simulink model "single_phase_to_3phase"  (R2025a)
settings: Solver=ode23tb  StartTime=0.0  StopTime=10.0  RelTol=1e-3  EnableMultiTasking=on
undefined symbols (not defined in the file): DiscIntNeverNeededParam, LowerLimit, UpperLimit, Vsrc_amp
libraries: powerlib_extras x8, spsVoltageMeasurementLib x7, spsGroundLib x5, spsSeriesRLCBranchLib x4, spsThreePhaseSeriesRLCBranchLib x2, spsUniversalBridgeLib x2, spsACVoltageSourceLib x1, simulink x1, spsThreePhaseSeriesRLCLoadLib x1, spsThreePhaseVIMeasurementLib x1, spspowerguiLib x1
settings Model: Creator=DELL  LastModifiedBy=SimuVerity Contributors
settings SolverCC: ZeroCrossAlgorithm=Non-adaptive  AlgebraicLoopSolver=TrustRegion
settings DataIOCC: LimitDataPoints=on  SaveFormat=Array  SignalLoggingSaveFormat=ModelDataLogs  ReturnWorkspaceOutputs=off
settings OptimizationCC: ExpressionDepthLimit=2147483647.0  InitFltsAndDblsToZero=on  LifeSpan=inf
settings DebuggingCC: UnderspecifiedInitializationDetection=Classic  MergeDetectMultiDrivingBlocksExec=none  SolverPrmCheckMsg=warning  FcnCallInpInsideContextMsg=warning  UnconnectedInputMsg=warning  UnconnectedOutputMsg=warning  UnconnectedLineMsg=warning  StateNameClashWarn=warning  SFUnexpectedBacktrackingDiag=warning  SFNoUnconditionalDefaultTransitionDiag=warning  SFExecutionAtInitializationDiag=none  ArithmeticOperatorsInVariantConditions=warning
settings HardwareCC: ProdBitPerPointer=32.0  ProdBitPerSizeT=32.0  ProdBitPerPtrDiffT=32.0  ProdLargestAtomicFloat=None  ProdIntDivRoundTo=Undefined  ProdEndianess=Unspecified  ProdWordSize=32.0  ProdHWDeviceType=32-bit Generic
settings ModelReferenceCC: PropagateSignalLabelsOutOfModel=off
settings RTWCC: GPUComputeCapability=3.5
settings CodeAppCC: StateflowObjectComments=on
settings GRTTargetCC: TargetLangStandard=C89/C90 (ANSI)  CombineOutputUpdateFcns=off  GRTInterface=on
settings ConfigComp: CovMetricSettings=dw  CovSaveCumulativeToWorkspaceVar=on  CovSaveSingleToWorkspaceVar=on

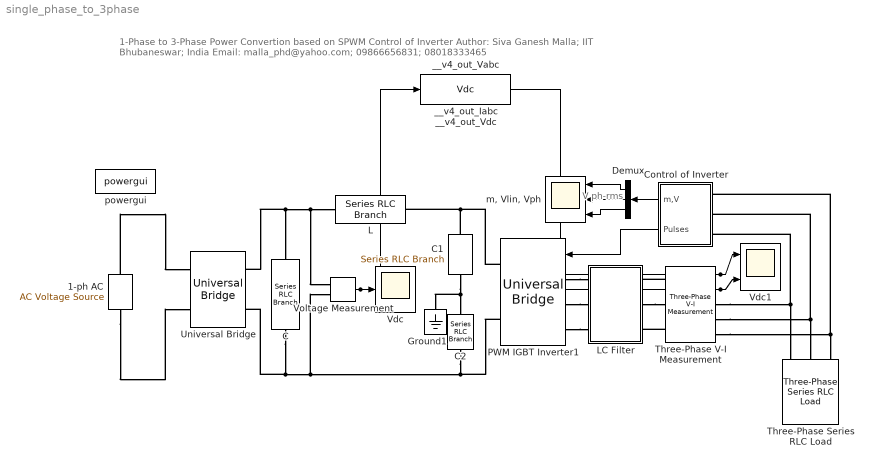
== system single_phase_to_3phase ==
  note: V ph-rms
  note: 1-Phase to 3-Phase Power Convertion based on SPWM Control of Inverter
      | Author: Siva Ganesh Malla; IIT Bhubaneswar; India
      | Email: malla_phd@yahoo.com; 09866656831; 08018333465
  1-ph AC : spsACVoltageSourceLib/AC Voltage Source  Amplitude=Vsrc_amp  Phase=0  Frequency=50  SampleTime=0.00001  Measurements=None  BusType=swing  Pref=10e3  Qref=0  Qmin=-inf  Qmax=+inf
  C : spsSeriesRLCBranchLib/Series RLC Branch  LConnTagsString=__new0  RConnTagsString=__new0  BranchType=C  Resistance=1  Inductance=1e-3  SetiL0=off  InitialCurrent=0  Capacitance=10e-6  Setx0=off  InitialVoltage=0  Measurements=None
  C1 : spsSeriesRLCBranchLib/Series RLC Branch  LConnTagsString=__new0  RConnTagsString=__new0  BranchType=C  Resistance=1  Inductance=1e-3  SetiL0=off  InitialCurrent=0  Capacitance=2300e-6  Setx0=off  InitialVoltage=0  Measurements=None
  C2 : spsSeriesRLCBranchLib/Series RLC Branch  LConnTagsString=__new0  RConnTagsString=__new0  BranchType=C  Resistance=1  Inductance=1e-3  SetiL0=off  InitialCurrent=0  Capacitance=2300e-6  Setx0=off  InitialVoltage=0  Measurements=None
  Control of Inverter : Subsystem
  Demux : Demux  Outputs=3
  Ground1 : spsGroundLib/Ground  LConnTagsString=a
  L : spsSeriesRLCBranchLib/Series RLC Branch  LConnTagsString=__new0  RConnTagsString=__new0  BranchType=L  Resistance=1  Inductance=0.1e-3  SetiL0=off  InitialCurrent=0  Capacitance=1e-6  Setx0=off  InitialVoltage=0  Measurements=None
  LC Filter : Subsystem
  PWM IGBT Inverter1 : spsUniversalBridgeLib/Universal Bridge  Arms=3  SnubberResistance=5000  SnubberCapacitance=inf  Device=GTO / Diodes  Ron=1e-3  Lon=0  ForwardVoltages="[  0.0  0.0  ]"  ForwardVoltage=.8  GTOparameters=[ 1e-6 ,1e-6 ]  IGBTparameters=[ 1e-6 , 2e-6 ]  Measurements=Device currents  Measurements_2=None  converterType=Rectifier
      settings: AttributesFormatString=\n
  Three-Phase Series RLC Load : spsThreePhaseSeriesRLCLoadLib/Three-Phase Series RLC Load  LConnTagsString=A|B|C  Configuration=Y (grounded)  NominalVoltage=400  Vabc=[1e3 1e3 1e3]  Vabcp=[1e3 1e3 1e3]  NominalFrequency=50  UnbalancedPower=off  ActivePower=P_load  InductivePower=0  CapacitivePower=0  Pabc=[10e3 9e3 11e3]  QLabc=[100 90 110]  QCabc=[100 90 110]  Pabcp=[10e3 9e3 11e3]  QLabcp=[100 90 110]  QCabcp=[100 90 110]  Measurements=None  LoadType=constant Z
  Three-Phase V-I Measurement : spsThreePhaseVIMeasurementLib/Three-Phase V-I Measurement  VoltageMeasurement=phase-to-ground  SetLabelV=off  LabelV=Vabc  Vpu=off  VpuLL=off  CurrentMeasurement=yes  SetLabelI=off  LabelI=Iabc  Ipu=off  Pbase=100e6  Vbase=500e3  OutputType=Complex  PhasorSimulation=off  PSBequivalent=0
  Universal Bridge : spsUniversalBridgeLib/Universal Bridge  Arms=2  SnubberResistance=1e5  SnubberCapacitance=inf  Device=Diodes  Ron=1e-3  Lon=0  ForwardVoltages="[  0  0  ]"  ForwardVoltage=0  GTOparameters=[ 10e-6 , 20e-6 ]  IGBTparameters=[ 1e-6 , 2e-6 ]  Measurements=None  Measurements_2=None  converterType=Rectifier
  Vdc : Scope
      settings: SampleTime=100e-6  TimeSpan=1  ActiveDisplayYMinimum=475  ActiveDisplayYMaximum=675  DataLoggingVariableName=Ia_1
  Vdc1 : Scope  NumInputPorts=2
      settings: SampleTime=100e-6  TimeSpan=1  ActiveDisplayYMinimum=-350  ActiveDisplayYMaximum=350  DataLoggingVariableName=Ia_2
  Voltage Measurement : spsVoltageMeasurementLib/Voltage Measurement  PhasorSimulation=off  OutputType=Complex  PSBequivalent=0
  __v4_out_Iabc : ToWorkspace  VariableName=Iabc  SaveFormat=Timeseries  SampleTime=-1
  __v4_out_Vabc : ToWorkspace  VariableName=Vabc  SaveFormat=Timeseries  SampleTime=-1
  __v4_out_Vdc : ToWorkspace  VariableName=Vdc  SaveFormat=Timeseries  SampleTime=-1
  "m, Vlin, Vph" : Scope  NumInputPorts=3
      settings: SampleTime=100e-6  TimeSpan=1  ActiveDisplayYMinimum=0.93  ActiveDisplayYMaximum=0.995  DataLoggingVariableName=Ia_
  powergui : spspowerguiLib/powergui  SimulationMode=Discrete  SampleTime=50e-6  frequency=60  Iterations=50  frequencyindice=0  Pbase=100e6  ErrMax=1e-4  UnitsV=kV  UnitsW=MW  buscounter=0  FunctionMessages=off  echomessages=off  EnableUseOfTLC=off  CurrentSourceSwitches=off  DisableSnubberDevices=off  DisableRonSwitches=off  DisableVfSwitches=off  DisplayEquations=off  AutomaticDiscreteSolvers=off  SolverType=Tustin/Backward Euler (TBE)  Interpol=off  ExternalGateDelay=off  methode=off  Ts=0  x0status=blocks  SPID=off  SwTol=0  HookPort=off  NonlinearTolerance=1e-4  nMaxIteration=100  ContinueOnMaxIteration=off  RestoreLinks=warning  ResistiveCurrentMeasurement=off  Frange=[0:2:500]  Ylog=off  Xlog=on  ShowGrid=off  save=off  variable=ZData  structure=0  ZoomFFT=on  StartTime=0.0  cycles=1  DisplayStyle=1  fundamental=60  FreqAxis=off  MaxFrequency=1000  frequencyindicesteady=1  RmsSteady=1  display=off
  wires:
  Control of Inverter/2(Pulses) -> PWM IGBT Inverter1/1
  Control of Inverter/1(m,V) -> Demux/1
  Demux/1 -> "m, Vlin, Vph"/1
  Demux/2 -> "m, Vlin, Vph"/2
  Demux/3 -> "m, Vlin, Vph"/3
  Voltage Measurement/1 -> Vdc/1, __v4_out_Vdc/1
  Three-Phase V-I Measurement/1 -> Vdc1/1, __v4_out_Vabc/1
  Three-Phase V-I Measurement/2 -> Vdc1/2, __v4_out_Iabc/1
  connections:
  1-ph AC/RConn1 -- Universal Bridge/LConn1
  1-ph AC/LConn1 -- Universal Bridge/LConn2
  Universal Bridge/RConn1 -- C/LConn1 -- L/LConn1 -- Voltage Measurement/LConn1
  Universal Bridge/RConn2 -- C/RConn1 -- C2/RConn1 -- PWM IGBT Inverter1/RConn2 -- Voltage Measurement/LConn2
  PWM IGBT Inverter1/LConn1 -- LC Filter/LConn1
  PWM IGBT Inverter1/LConn2 -- LC Filter/LConn2
  PWM IGBT Inverter1/LConn3 -- LC Filter/LConn3
  Three-Phase V-I Measurement/RConn1 -- Three-Phase Series RLC Load/LConn1 -- Control of Inverter/LConn3
  Three-Phase V-I Measurement/RConn2 -- Three-Phase Series RLC Load/LConn2 -- Control of Inverter/LConn2
  Three-Phase V-I Measurement/RConn3 -- Three-Phase Series RLC Load/LConn3 -- Control of Inverter/LConn1
  Three-Phase V-I Measurement/LConn1 -- LC Filter/RConn1
  LC Filter/RConn2 -- Three-Phase V-I Measurement/LConn2
  Three-Phase V-I Measurement/LConn3 -- LC Filter/RConn3
  C1/LConn1 -- PWM IGBT Inverter1/RConn1 -- L/RConn1
  C1/RConn1 -- C2/LConn1 -- Ground1/LConn1

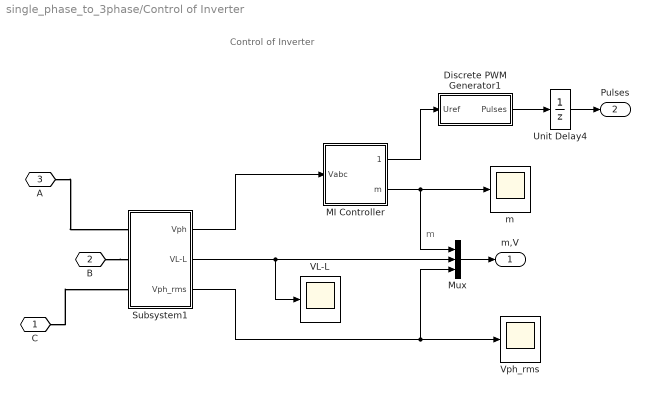
== system single_phase_to_3phase/Control of Inverter ==
  note: Control of Inverter
  note: m
  Discrete PWM Generator1 : Subsystem  AncestorBlock=|  DialogController=POWERSYS.PowerSysDialog  mask(Discrete PWM Generator){GeneratorMode=3-arm  bridge (6 pulses), Fc=4000, Ts=20e-6, Internal=off, mIndex=0.95, Freq=50, Phase=0}
      | powerlib_extras/Discrete 
      | Control Blocks/Discrete
      | PWM Generator
      mask prompts: GeneratorMode "Generator Mode"; Fc "Carrier frequency (Hz):"; Ts "Sample time:"; Internal "Internal generation of modulating signal(s)"; mIndex "Modulation index  (0<m<1) :"; Freq "Frequency of output voltage (Hz)"; Phase "Phase of output voltage (degrees)"
      mask help:
      | This discrete block generates pulses for carrier-based PWM (Pulse Width Modulation), self-commutated IGBTs,GTOs or FETs bridges.
      |
      | Depending on the number of bridge arms selected in the "Generator Mode" parameter, the block can be used either for single-phase or three-phase PWM control.
      mask init:
      | powericon('psbcallbacks',gcb,'Discrete PWM Generator');
      | if Freq==0
      |     Phase=90;
      | end
      | switch GeneratorMode
      | case 1,
      |     Internal_Phase=0;
      |    Signal_PortWidth=1;
      |    Select1_Elements=[1 2];
      |    Select1_PortWidth=2;
      |    Select3_Elements=[1 2];
      |    Select3_PortWidth=4;
      | case 2,
      |     Internal_Phase=0;
      |     Signal_PortWidth=1;
      |     Select1_Elements=[1 2];
      |     Select1_PortWidth=2;
      |     Select3_Elements=[1 2 3 4];
      |     Select3_PortWidth=4;
      | case 3,
      |     Internal_Phase=[0 -2*pi/3 2*pi/3];
      |     Signal_PortWidth=3;
      |     Select1_Elements=[1 4 2 5 3 6];
      |     Select1_PortWidth=6;
      |    Select3_Elements=[1 2 3 4 5 6];
      |    Select3_PortWidth=12;
      | case 4,
      |     Internal_Phase=[0 -2*pi/3 2*pi/3];
      |     Signal_PortWidth=3;
      |     Select1_Elements=[1 4 2 5 3 6];
      |     Select1_PortWidth=6;
      |    Select3_Elements=[1 2 3 4 5 6 7 8 9 10 11 12];
      |    Select3_PortWidth=12;
      | end
      | power_initmask();
      mask Help:
      | The output pulses are a vector (with values=0 or 1). Depending on the selected "Generator Mode", the output vector contains:
      | For a 1-arm  bridge: Two pulses. Pulse 1 is for the upper switch and pulse 2 is for the lower switch.
      | For a 2-arm  bridge: Four pulses. Pulses 1 and 3 are respectively for the upper switches of the first and second arm. Pulses 2 and 4 are for the lower switches.
      | For a 3-arm  bridge: Six pulses. Pulses 1,3 and 5 are respectively for the upper switches of the first,second and third arm. Pulses 2,4 and 6 are for the lower switches.
      | For double 3-arm bridges: Twelve pulses.The first six pulses (pulses 1 to 6) must be sent to the first 3-arm bridge and the last six (pulses 7 to 12) to the second 3-arm bridge.
      | 
      | By selecting "Internal generation" you can can control the modulation index m, frequency and phase of the output voltage  from the internal parameters (m, Freq and Phase). Otherwise, external signals are used for pulse generation. The width of the input vector must be 1 for single phase bridges ( 1-arm or 2-arm)  and 3 for 3-phase bridges  (single or double bridge).
      mask TypeOptions GeneratorMode: 1-arm  bridge (2 pulses) | 2-arm  bridge (4 pulses) | 3-arm  bridge (6 pulses) | Double 3-arm  bridges (12 pulses)
      mask Callback Internal: powericon('psbcallbacks',gcb,'Discrete PWM Generator',[]);
  MI Controller : Subsystem
  Mux : Mux  Inputs=3
  Subsystem1 : Subsystem
  Unit Delay4 : UnitDelay  SampleTime=20e-6
  VL-L : Scope
      settings: SampleTime=100e-6  TimeSpan=0.4  ActiveDisplayYMinimum=-700  ActiveDisplayYMaximum=700  DataLoggingVariableName=Vabc_line
  Vph_rms : Scope
      settings: SampleTime=100e-6  TimeSpan=0.4  ActiveDisplayYMinimum=29.5  ActiveDisplayYMaximum=33.75  DataLoggingVariableName=Vabc_rms
  m : Scope
      settings: SampleTime=100e-6  TimeSpan=0.04  ActiveDisplayYMinimum=0.7  ActiveDisplayYMaximum=1.5  DataLoggingVariableName=modulation_index
  C : PMIOPort  Side=Left
  B : PMIOPort  Port=2  Side=Left
  A : PMIOPort  Port=3  Side=Left
  m,V : Outport
  Pulses : Outport  Port=2
  wires:
  Mux/1 -> m,V/1
  MI Controller/2(m) -> m/1, Mux/1
  Unit Delay4/1 -> Pulses/1
  Discrete PWM Generator1/1(Pulses) -> Unit Delay4/1
  MI Controller/1(Vabc_inv) -> Discrete PWM Generator1/1(Uref)
  Subsystem1/1(Vph) -> MI Controller/1(Vabc)
  Subsystem1/2(VL-L) -> VL-L/1, Mux/2
  Subsystem1/3(Vph_rms) -> Vph_rms/1, Mux/3
  connections:
  A/RConn1 -- Subsystem1/LConn1
  B/RConn1 -- Subsystem1/LConn2
  C/RConn1 -- Subsystem1/LConn3

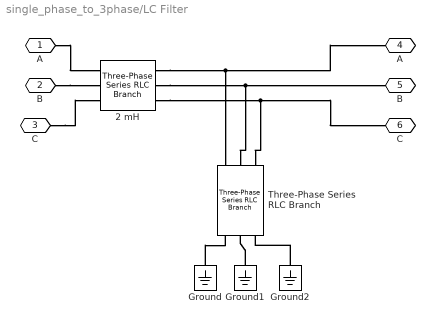
== system single_phase_to_3phase/LC Filter ==
  "2 mH " : spsThreePhaseSeriesRLCBranchLib/Three-Phase Series RLC Branch  LConnTagsString=A|B|C  RConnTagsString=A|B|C  BranchType=L  Resistance=1.0  Inductance=36e-3  Capacitance=1.0  Measurements=None
  Ground : spsGroundLib/Ground  LConnTagsString=a
  Ground1 : spsGroundLib/Ground  LConnTagsString=a
  Ground2 : spsGroundLib/Ground  LConnTagsString=a
  Three-Phase Series RLC Branch : spsThreePhaseSeriesRLCBranchLib/Three-Phase Series RLC Branch  LConnTagsString=A|B|C  RConnTagsString=A|B|C  BranchType=C  Resistance=.1  Inductance=1e-3  Capacitance=6.85e-7  Measurements=None
  A : PMIOPort  Side=Left
  B : PMIOPort  Port=2  Side=Left
  C : PMIOPort  Port=3  Side=Left
  "A " : PMIOPort  Port=4  Side=Right
  "B " : PMIOPort  Port=5  Side=Right
  "C " : PMIOPort  Port=6  Side=Right
  connections:
  B/RConn1 -- "2 mH "/LConn2
  A/RConn1 -- "2 mH "/LConn1
  C/RConn1 -- "2 mH "/LConn3
  "2 mH "/RConn1 -- "A "/RConn1 -- Three-Phase Series RLC Branch/LConn1
  "2 mH "/RConn2 -- "B "/RConn1 -- Three-Phase Series RLC Branch/LConn2
  "2 mH "/RConn3 -- "C "/RConn1 -- Three-Phase Series RLC Branch/LConn3
  Ground/LConn1 -- Three-Phase Series RLC Branch/RConn1
  Ground1/LConn1 -- Three-Phase Series RLC Branch/RConn2
  Ground2/LConn1 -- Three-Phase Series RLC Branch/RConn3

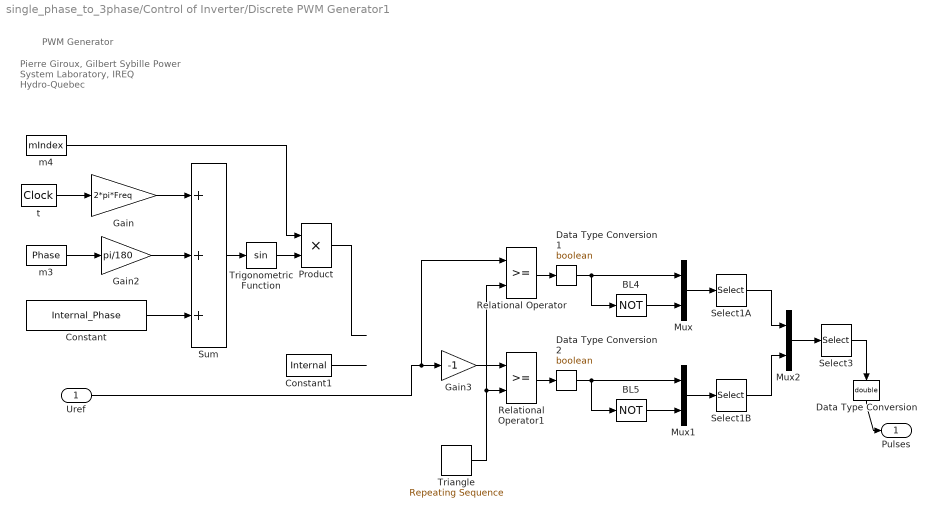
== system single_phase_to_3phase/Control of Inverter/Discrete PWM Generator1 ==
  note: Pierre Giroux, Gilbert Sybille
      | Power System Laboratory, IREQ
      | Hydro-Quebec
  note: PWM Generator
  Uref : Inport
  BL4 : Logic  Operator=NOT  Inputs=1
  BL5 : Logic  Operator=NOT  Inputs=1
  Constant : Constant  Value=Internal_Phase
  Constant1 : Constant  Value=Internal
  Data Type Conversion : DataTypeConversion  OutDataTypeStr=double
  Data Type Conversion1 : DataTypeConversion  OutDataTypeStr=boolean
  Data Type Conversion2 : DataTypeConversion  OutDataTypeStr=boolean
  Gain : Gain  Gain=2*pi*Freq  SaturateOnIntegerOverflow=on  OutDataTypeStr=Inherit: Same as input  ParamDataTypeStr=Inherit: Same as input
  Gain2 : Gain  Gain=pi/180  SaturateOnIntegerOverflow=on  OutDataTypeStr=Inherit: Same as input  ParamDataTypeStr=Inherit: Same as input
  Gain3 : Gain  Gain=-1  SaturateOnIntegerOverflow=on  OutDataTypeStr=Inherit: Same as input  ParamDataTypeStr=Inherit: Same as input
  Mux : Mux  Inputs=2
  Mux1 : Mux  Inputs=2
  Mux2 : Mux  Inputs=2
  Product : Product  InputSameDT=on  SaturateOnIntegerOverflow=on  OutDataTypeStr=Inherit: Same as first input
  Relational Operator : RelationalOperator
  Relational Operator1 : RelationalOperator
  Select1A : Selector  InputPortWidth=Select1_PortWidth  IndexOptions=Index vector (dialog)  Indices=Select1_Elements  OutputSizes=1
  Select1B : Selector  InputPortWidth=Select1_PortWidth  IndexOptions=Index vector (dialog)  Indices=Select1_Elements  OutputSizes=1
  Select3 : Selector  InputPortWidth=Select3_PortWidth  IndexOptions=Index vector (dialog)  Indices=Select3_Elements  OutputSizes=1
  Sum : Sum  Inputs=+++  InputSameDT=on  SaturateOnIntegerOverflow=on  OutDataTypeStr=Inherit: Same as first input
  Triangle : simulink/Sources/Repeating Sequence  rep_seq_t=[0 1/Fc/4 3/Fc/4 1/Fc]  rep_seq_y=[0 -1 1 0]
  Trigonometric Function : Trigonometry
  m3 : Constant  Value=Phase
  m4 : Constant  Value=mIndex
  t : DigitalClock  SampleTime=Ts
  Pulses : Outport
  wires:
  Mux2/1 -> Select3/1
  Select1B/1 -> Mux2/2
  Select1A/1 -> Mux2/1
  Mux1/1 -> Select1B/1
  Mux/1 -> Select1A/1
  BL5/1 -> Mux1/2
  BL4/1 -> Mux/2
  Gain3/1 -> Relational Operator1/1
  Triangle/1 -> Relational Operator1/2, Relational Operator/2
  Product/1 -> ?
  Constant1/1 -> ?
  Uref/1 -> Relational Operator/1, Gain3/1
  Trigonometric Function/1 -> Product/2
  Sum/1 -> Trigonometric Function/1
  m4/1 -> Product/1
  Constant/1 -> Sum/3
  m3/1 -> Gain2/1
  Gain2/1 -> Sum/2
  Gain/1 -> Sum/1
  t/1 -> Gain/1
  Select3/1 -> Data Type Conversion/1
  Data Type Conversion/1 -> Pulses/1
  Relational Operator/1 -> Data Type Conversion1/1
  Data Type Conversion1/1 -> BL4/1, Mux/1
  Relational Operator1/1 -> Data Type Conversion2/1
  Data Type Conversion2/1 -> BL5/1, Mux1/1

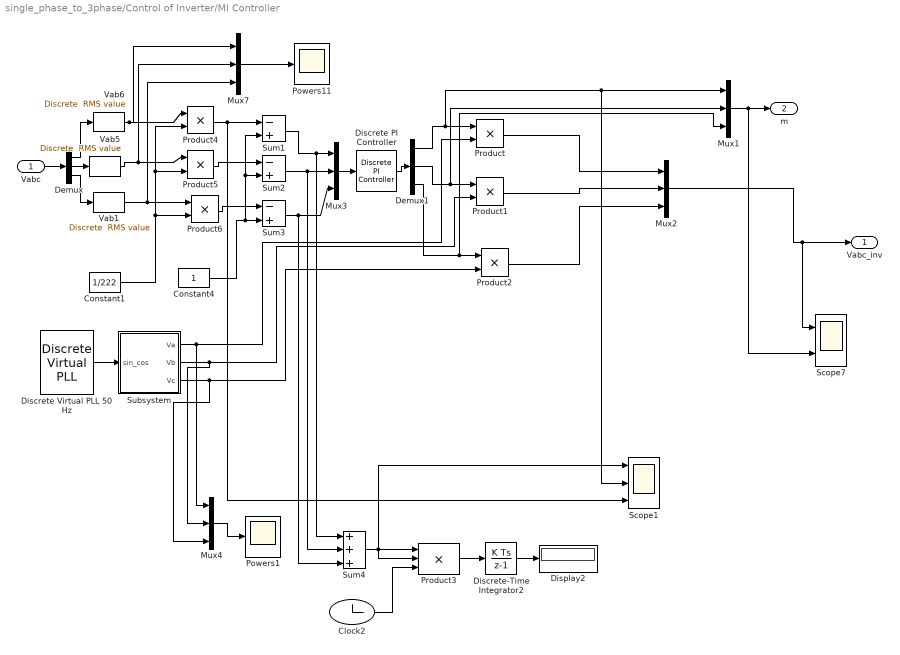
== system single_phase_to_3phase/Control of Inverter/MI Controller ==
  Vabc : Inport
  Clock2 : Clock
  Constant1 : Constant  Value=1/222
  Constant4 : Constant
  Demux : Demux  Outputs=3
  Demux1 : Demux  Outputs=3
  Discrete PI Controller : powerlib_extras/Discrete  Control Blocks/Discrete PI Controller  Kp=1.6  Ki=36  Par_Limits=[1.2 -1]  Init=0  Ts=20e-6
  Discrete Virtual PLL 50 Hz : powerlib_extras/Discrete  Control Blocks/Discrete Virtual PLL  Freq=50  Phase=0  Ts=20e-6
  Discrete-Time Integrator2 : DiscreteIntegrator  SampleTime=20e-6  UpperSaturationLimit=UpperLimit  LowerSaturationLimit=LowerLimit  ICPrevOutput=DiscIntNeverNeededParam  ICPrevScaledInput=DiscIntNeverNeededParam
  Display2 : Display
  Mux{1..4,7} (5 alike) : Mux  Inputs=3
  Powers1 : Scope
      settings: SampleTime=100e-6  ActiveDisplayYMinimum=-1  ActiveDisplayYMaximum=1  DataLoggingVariableName=ScopeData3
  Powers11 : Scope
      settings: SampleTime=100e-6  ActiveDisplayYMinimum=452  ActiveDisplayYMaximum=465  DataLoggingVariableName=ScopeData6
  Product{,1..2,4..6} (6 alike) : Product  RndMeth=Zero
  Product3 : Product  Inputs=3  InputSameDT=on  RndMeth=Zero  SaturateOnIntegerOverflow=on  OutDataTypeStr=Inherit: Same as first input
  Scope1 : Scope  NumInputPorts=3
      settings: TimeSpan=0.1  ActiveDisplayYMinimum=-0.005  ActiveDisplayYMaximum=0.0175  DataLoggingVariableName=psbbridges_str6
  Scope7 : Scope  NumInputPorts=2
      settings: TimeSpan=0.1  ActiveDisplayYMinimum=-1.1  ActiveDisplayYMaximum=1.1  DataLoggingVariableName=psbbridges_str2
  Subsystem : Subsystem
  Sum1 : Sum  Inputs=-+  InputSameDT=on  SaturateOnIntegerOverflow=on  OutDataTypeStr=Inherit: Same as first input
  Sum2 : Sum  Inputs=-+  InputSameDT=on  SaturateOnIntegerOverflow=on  OutDataTypeStr=Inherit: Same as first input
  Sum3 : Sum  Inputs=-+  InputSameDT=on  SaturateOnIntegerOverflow=on  OutDataTypeStr=Inherit: Same as first input
  Sum4 : Sum  Inputs=+++  InputSameDT=on  SaturateOnIntegerOverflow=on  OutDataTypeStr=Inherit: Same as first input
  Vab1 : powerlib_extras/Discrete Measurements/Discrete  RMS value  Freq=50  Mag_Init=0  Ts=20e-6
  Vab5 : powerlib_extras/Discrete Measurements/Discrete  RMS value  Freq=50  Mag_Init=0  Ts=20e-6
  Vab6 : powerlib_extras/Discrete Measurements/Discrete  RMS value  Freq=50  Mag_Init=0  Ts=20e-6
  Vabc_inv : Outport
  m : Outport  Port=2
  wires:
  Mux2/1 -> Vabc_inv/1, Scope7/1
  Product/1 -> Mux2/1
  Product1/1 -> Mux2/2
  Product2/1 -> Mux2/3
  Mux1/1 -> m/1, Scope7/2
  Vab5/1 -> Mux7/2, Product5/1
  Vab1/1 -> Mux7/3, Product6/1
  Constant4/1 -> Sum3/2, Sum2/2, Sum1/2
  Sum1/1 -> Mux3/1, Sum4/1
  Vabc/1 -> Demux/1
  Demux/1 -> Vab6/1
  Demux/2 -> Vab5/1
  Demux/3 -> Vab1/1
  Product3/1 -> Discrete-Time Integrator2/1
  Clock2/1 -> Product3/3
  Discrete-Time Integrator2/1 -> Display2/1
  Sum2/1 -> Mux3/2, Sum4/2
  Sum3/1 -> Mux3/3, Sum4/3
  Mux3/1 -> Discrete PI Controller/1
  Discrete PI Controller/1 -> Demux1/1
  Demux1/1 -> Product/1, Mux1/1, Scope1/2
  Demux1/2 -> Product1/1, Mux1/2
  Demux1/3 -> Product2/1, Mux1/3
  Product4/1 -> Sum1/1, Scope1/3
  Product5/1 -> Sum2/1
  Product6/1 -> Sum3/1
  Vab6/1 -> Mux7/1, Product4/1
  Mux7/1 -> Powers11/1
  Discrete Virtual PLL 50 Hz/2 -> Subsystem/1(sin_cos)
  Subsystem/1(Va) -> Product/2, Mux4/1
  Subsystem/2(Vb) -> Product1/2, Mux4/2
  Subsystem/3(Vc) -> Product2/2, Mux4/3
  Mux4/1 -> Powers1/1
  Constant1/1 -> Product6/2, Product5/2, Product4/2
  Sum4/1 -> Product3/1, Product3/2, Scope1/1

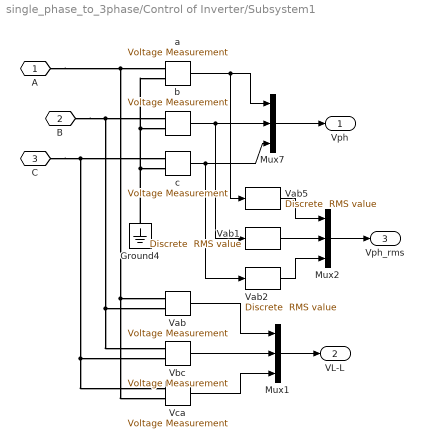
== system single_phase_to_3phase/Control of Inverter/Subsystem1 ==
  Ground4 : spsGroundLib/Ground  LConnTagsString=a
  Mux1 : Mux  Inputs=3
  Mux2 : Mux  Inputs=3
  Mux7 : Mux  Inputs=3
  Vab : spsVoltageMeasurementLib/Voltage Measurement  Tag=PoWeRsYsTeMmEaSuReMeNt  PhasorSimulation=off  OutputType=Magnitude  PSBequivalent=0
  Vab1 : powerlib_extras/Discrete Measurements/Discrete  RMS value  Freq=50  Mag_Init=0  Ts=20e-6
  Vab2 : powerlib_extras/Discrete Measurements/Discrete  RMS value  Freq=50  Mag_Init=0  Ts=20e-6
  Vab5 : powerlib_extras/Discrete Measurements/Discrete  RMS value  Freq=50  Mag_Init=0  Ts=20e-6
  Vbc : spsVoltageMeasurementLib/Voltage Measurement  Tag=PoWeRsYsTeMmEaSuReMeNt  PhasorSimulation=off  OutputType=Magnitude  PSBequivalent=0
  Vca : spsVoltageMeasurementLib/Voltage Measurement  Tag=PoWeRsYsTeMmEaSuReMeNt  PhasorSimulation=off  OutputType=Magnitude  PSBequivalent=0
  a : spsVoltageMeasurementLib/Voltage Measurement  Tag=PoWeRsYsTeMmEaSuReMeNt  PhasorSimulation=off  OutputType=Magnitude  PSBequivalent=0
  b : spsVoltageMeasurementLib/Voltage Measurement  Tag=PoWeRsYsTeMmEaSuReMeNt  PhasorSimulation=off  OutputType=Magnitude  PSBequivalent=0
  c : spsVoltageMeasurementLib/Voltage Measurement  Tag=PoWeRsYsTeMmEaSuReMeNt  PhasorSimulation=off  OutputType=Magnitude  PSBequivalent=0
  A : PMIOPort  Side=Left
  B : PMIOPort  Port=2  Side=Left
  C : PMIOPort  Port=3  Side=Left
  Vph : Outport
  VL-L : Outport  Port=2
  Vph_rms : Outport  Port=3
  wires:
  a/1 -> Mux7/1, Vab5/1
  b/1 -> Mux7/2, Vab1/1
  c/1 -> Mux7/3, Vab2/1
  Mux7/1 -> Vph/1
  Vab/1 -> Mux1/1
  Vbc/1 -> Mux1/2
  Vca/1 -> Mux1/3
  Mux1/1 -> VL-L/1
  Vab5/1 -> Mux2/1
  Vab1/1 -> Mux2/2
  Vab2/1 -> Mux2/3
  Mux2/1 -> Vph_rms/1
  connections:
  Ground4/LConn1 -- c/LConn2 -- b/LConn2 -- a/LConn2
  A/RConn1 -- a/LConn1 -- Vab/LConn1 -- Vca/LConn2
  B/RConn1 -- b/LConn1 -- Vab/LConn2 -- Vbc/LConn1
  C/RConn1 -- c/LConn1 -- Vbc/LConn2 -- Vca/LConn1

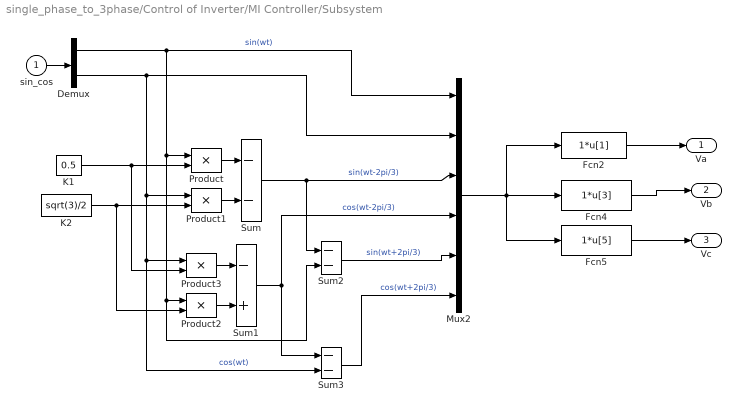
== system single_phase_to_3phase/Control of Inverter/MI Controller/Subsystem ==
  sin_cos : Inport  PortDimensions=2
  Demux : Demux  Outputs=2
      settings: DisplayOption=none
  Fcn2 : Fcn  Expr=1*u[1]
  Fcn4 : Fcn  Expr=1*u[3]
  Fcn5 : Fcn  Expr=1*u[5]
  K1 : Constant  Value=0.5
  K2 : Constant  Value=sqrt(3)/2
  Mux2 : Mux  Inputs=6
  Product{,1..3} (4 alike) : Product  InputSameDT=on  SaturateOnIntegerOverflow=on  OutDataTypeStr=Inherit: Same as first input
  Sum : Sum  Inputs=--  InputSameDT=on  SaturateOnIntegerOverflow=on  OutDataTypeStr=Inherit: Same as first input
  Sum1 : Sum  Inputs=-+  InputSameDT=on  SaturateOnIntegerOverflow=on  OutDataTypeStr=Inherit: Same as first input
  Sum2 : Sum  Inputs=--  InputSameDT=on  SaturateOnIntegerOverflow=on  OutDataTypeStr=Inherit: Same as first input
  Sum3 : Sum  Inputs=--  InputSameDT=on  SaturateOnIntegerOverflow=on  OutDataTypeStr=Inherit: Same as first input
  Va : Outport
  Vb : Outport  Port=2
  Vc : Outport  Port=3
  wires:
  sin_cos/1 -> Demux/1
  Demux/1 -> Product/1, Product2/1, Sum2/2, Mux2/1  "sin(wt)"
  Product/1 -> Sum/1
  Product1/1 -> Sum/2
  Product3/1 -> Sum1/1
  Product2/1 -> Sum1/2
  Sum3/1 -> Mux2/6  "cos(wt+2pi/3)"
  Sum2/1 -> Mux2/5  "sin(wt+2pi/3)"
  K1/1 -> Product/2, Product3/2
  K2/1 -> Product1/2, Product2/2
  Sum/1 -> Mux2/3, Sum2/1  "sin(wt-2pi/3)"
  Sum1/1 -> Mux2/4, Sum3/1  "cos(wt-2pi/3)"
  Demux/2 -> Sum3/2, Product3/1, Product1/1, Mux2/2  "cos(wt)"
  Mux2/1 -> Fcn2/1, Fcn4/1, Fcn5/1
  Fcn2/1 -> Va/1
  Fcn4/1 -> Vb/1
  Fcn5/1 -> Vc/1
